simulink model "mars_rover_test_harness_chassis"  (R2025a)
settings: Solver=ode23t  StartTime=0.0  StopTime=30  FixedStep=1e-10  MaxStep=1e-1  RelTol=1e-3  AbsTol=1e-3  EnableMultiTasking=on
undefined symbols (not defined in the file): arm_q0, Control, L1, L2, L3, LS1, LS3, R1, R2, R3, Rover, RS1, RS3, X, Y, Z
libraries: sm_lib x119, nesl_utility x99, fl_lib x85, sdl_lib x20, ee_lib x10, mars_rover_lib x8, simulink x5, slpidlib x3, batteryecm_lib x2
(part 1 of 8)
Description:
  | Mars Rover Chassis Test Harness
  | Copyright 2022-2025 The MathWorks, Inc.
settings Model: VariantFading=off  Creator=The MathWorks, Inc.  LastModifiedBy=smiller
settings SolverCC: AutoScaleAbsTol=off  MaxConsecutiveZCs=500  AlgebraicLoopSolver=TrustRegion  MinimalZcImpactIntegration=on
settings DataIOCC: MaxDataPoints=10000  SaveFormat=Array  ReturnWorkspaceOutputs=off  SignalLoggingName=logsout_mars_rover_terrain
settings OptimizationCC: ReuseModelBlockBuffer=off  LifeSpan=inf
settings DebuggingCC: UnconnectedInputMsg=warning  UnconnectedOutputMsg=warning  UnconnectedLineMsg=warning  AllowSymbolicDim=off  SFUnexpectedBacktrackingDiag=warning  SFNoUnconditionalDefaultTransitionDiag=warning  SFExecutionAtInitializationDiag=none  ArithmeticOperatorsInVariantConditions=warning
settings ModelReferenceCC: EnableRefExpFcnMdlSchedulingChecks=on
settings SFSimCC: SimUseLocalCustomCode=off  CustomCodeUndefinedFunction=UseInterfaceOnly
settings RTWCC: RTWUseLocalCustomCode=off  GPUComputeCapability=3.5  DLArmComputeVersion=19.05
settings CodeAppCC: StateflowObjectComments=on
settings GRTTargetCC: TargetLangStandard=C89/C90 (ANSI)
settings ConfigComp: CovMetricSettings=dw  CovSaveCumulativeToWorkspaceVar=on  CovSaveSingleToWorkspaceVar=on  CovExternalEMLEnable=off  CovSFcnEnable=off
settings SimscapeCC: SimscapeLogType=all  SimscapeLogSimulationStatistics=on  SimscapeLogName=simlog_mars_rover_terrain  SimscapeLogLimitData=off  SimscapeLogDataHistory=10000.0  SimscapeOperatingPoint=sm_mars_rover_op
settings DiagnosticsConfigSet: SimMechanicsUnconnectedFramePorts=none  SimMechanicsConflictingReferenceFrames=none
settings ExplorerConfigSet: InternalSimMechanicsExplorerSettings="<ExplorerConfiguration><canonicalview>default</canonicalview><AnimationSetting><BasePlaybackSpeed>1.0</BasePlaybackSpeed><PlaybackSpeedFactor>2.0</PlaybackSpeedFactor></AnimationSetting><TilePanel><TileInfo><Tiles Columns=\"2\" Count=\"2\" Rows=\"1\"><Column Weight=\"0.5621\"/><Column Weight=\"0.4379\"/><Row Weight=\"1\"/><Tile Height=\"1\" Width=\"1\" X=\"0\" Y=\"0\"/><Tile Height=\"1\" Width=\"1\" X=\"1\" Y=\"0\"/></Tiles></TileInfo><SceneInfo><SceneViewer><BGColor><R>1</R><G>1</G><B>1</B></BGColor><Camera><DoPerspective>off</DoPerspective><Position><X>0.0384762068557005787</X><Y>-1.89513590882941751</Y><Z>0.280552334311850116</Z></Position><Center><X>0.0384762068557005787</X><Y>3.68387699789529677e-08</Y><Z>0.280552334311850116</Z></Center><Up><X>0</X><Y>-0</Y><Z>1</Z></Up><ViewLimDist>1</ViewLimDist><YLim>1.19054091853124122</YLim><XLim>1.46367727637290956</XLim></Camera></SceneViewer><SceneViewer><BGColor><R>1</R><G>1</G><B>1</B></BGColor><Camera><DoPerspective>off</DoPerspective><Position><X>0.0374473281726132104</X><Y>-0.000143741231528847491</Y><Z>2.19998367982950649</Z></Position><Center><X>0.0374473281726132104</X><Y>-0.000143741231528847491</Y><Z>0.280552368074773462</Z></Center><Up><X>0.999998749919673302</X><Y>0.00158118913824325125</Y><Z>0</Z></Up><ViewLimDist>1</ViewLimDist><YLim>1.46318539738655096</YLim><XLim>1.39912298944493307</XLim></Camera></SceneViewer></SceneInfo></TilePanel><MechEditorPanel><Cameras><Camera><Id>Camera7</Id><Value><Name>Chassis_Rear</Name><NativeCamera><PositionTrackingFeature>Rover.Chassis.Chassis.Camera_Frames.Reference_Chassis_Camera_Rear.R</PositionTrackingFeature><CenterTrackingFeature>Rover.Chassis.Chassis.Camera_Frames.Reference_Chassis_Camera_Rear.R</CenterTrackingFeature><UpVectorTrackingFeature>Rover.World_Frame.W</UpVectorTrackingFeature><CenterTrackingOrigin>off</CenterTrackingOrigin><CenterTrackingDirection>-Y</CenterTrackingDirection><UpVectorTrackingDirection>+Z</UpVectorTrackingDirection></NativeCamera></Value></Camera><Camera><Id>Camera8</Id><Value><Name>Chassis_Right</Name><NativeCamera><PositionTrackingFeature>Rover.Chassis.Chassis.Camera_Frames.Reference_Chassis_Camera_Right.R</PositionTrackingFeature><CenterTrackingFeature>Rover.Chassis.Chassis.Camera_Frames.Reference_Chassis_Camera_Right.R</CenterTrackingFeature><UpVectorTrackingFeature>Rover.World_Frame.W</UpVectorTrackingFeature><CenterTrackingOrigin>off</CenterTrackingOrigin><CenterTrackingDirection>+X</CenterTrackingDirection><UpVectorTrackingDirection>+Z</UpVectorTrackingDirection></NativeCamera></Value></Camera><Camera><Id>Camera9</Id><Value><Name>Chassis_Top</Name><NativeCamera><PositionTrackingFeature>Rover.Chassis.Chassis.Camera_Frames.Reference_Chassis_Camera_Top.R</PositionTrackingFeature><CenterTrackingFeature>Rover.Chassis.Chassis.Camera_Frames.Reference_Chassis_Camera_Top.R</CenterTrackingFeature><UpVectorTrackingFeature>Rover.World_Frame.W</UpVectorTrackingFeature><CenterTrackingOrigin>off</CenterTrackingOrigin><CenterTrackingDirection>-Z</CenterTrackingDirection><UpVectorTrackingDirection>+Y</UpVectorTrackingDirection></NativeCamera></Value></Camera><Camera><Id>Camera10</Id><Value><Name>Whl_L1</Name><NativeCamera><PositionTrackingFeature>Rover.Chassis.Roll_and_Steer.Drive.Camera_Frame_L1.Reference_Cam_Whl.R</PositionTrackingFeature><CenterTrackingFeature>Rover.Chassis.Roll_and_Steer.Drive.Camera_Frame_L1.Reference_Cam_Whl.R</CenterTrackingFeature><UpVectorTrackingFeature>Rover.Chassis.Roll_and_Steer.Drive.Camera_Frame_L1.Reference_Cam_Whl.R</UpVectorTrackingFeature><CenterTrackingOrigin>off</CenterTrackingOrigin><CenterTrackingDirection>-Z</CenterTrackingDirection><UpVectorTrackingDirection>+X</UpVectorTrackingDirection></NativeCamera></Value></Camera><Camera><Id>Camera11</Id><Value><Name>Whl_R1</Name><NativeCamera><PositionTrackingFeature>Rover.Chassis.Roll_and_Steer.Drive.Camera_Frame_R1.Reference_Cam_Whl.R</PositionTrackingFeature><CenterTrackingFeature>Rover.Chassis.Roll_and_Steer.Drive.Camera_Frame_R1.Reference_Cam_Whl.R</CenterTrackingFeature><UpVectorTrackingFeature>Rover.Chassis.Roll_and_Steer.Drive.Camera_Frame_R1.Reference_Cam_Whl.R</UpVectorTrackingFeature><CenterTrackingOrigin>off</CenterTrackingOrigin><CenterTrackingDirection>+Z</CenterTrackingDirection><UpVectorTrackingDirection>-X</UpVectorTrackingDirection></NativeCamera></Value></Camera><Camera><Id>Camera12</Id><Value><Name>Whl_L2</Name><NativeCamera><PositionTrackingFeature>Rover.Chassis.Roll_and_Steer.Drive.Camera_Frame_L2.Reference_Cam_Whl.R</PositionTrackingFeature><CenterTrackingFeature>Rover.Chassis.Roll_and_Steer.Drive.Camera_Frame_L2.Reference_Cam_Whl.R</CenterTrackingFeature><UpVectorTrackingFeature>Rover.Chassis.Roll_and_Steer.Drive.Camera_Frame_L2.Reference_Cam_Whl.R</UpVectorTrackingFeature><CenterTrackingOrigin>off</CenterTrackingOrigin><CenterTrackingDirection>-Z</CenterTrackingDirection><UpVectorTrackingDirection>-Y</UpVectorTrackingDirection></NativeCamera></Value></Camera><Camera><Id>Camera13</Id><Value><Name>Whl_R2</Name><NativeCamera><PositionTrackingFeature>Rover.Chassis.Roll_and_Steer.Drive.Camera_Frame_R2.Reference_Cam_Whl.R</PositionTrackingFeature><CenterTrackingFeature>Rover.Chassis.Roll_and_Steer.Drive.Camera_Frame_R2.Reference_Cam_Whl.R</CenterTrackingFeature><UpVectorTrackingFeature>Rover.Chassis.Roll_and_Steer.Drive.Camera_Frame_R2.Reference_Cam_Whl.R</UpVectorTrackingFeature><CenterTrackingOrigin>off</CenterTrackingOrigin><CenterTrackingDirection>+Z</CenterTrackingDirection><UpVectorTrackingDirection>+Y</UpVectorTrackingDirection></NativeCamera></Value></Camera><Camera><Id>Camera14</Id><Value><Name>Whl_L3</Name><NativeCamera><PositionTrackingFeature>Rover.Chassis.Roll_and_Steer.Drive.Camera_Frame_L3.Reference_Cam_Whl.R</PositionTrackingFeature><CenterTrackingFeature>Rover.Chassis.Roll_and_Steer.Drive.Camera_Frame_L3.Reference_Cam_Whl.R</CenterTrackingFeature><UpVectorTrackingFeature>Rover.Chassis.Roll_and_Steer.Drive.Camera_Frame_L3.Reference_Cam_Whl.R</UpVectorTrackingFeature><CenterTrackingOrigin>off</CenterTrackingOrigin><CenterTrackingDirection>-Z</CenterTrackingDirection><UpVectorTrackingDirection>+X</UpVectorTrackingDirection></NativeCamera></Value></Camera><Camera><Id>Camera15</Id><Value><Name>Whl_R3</Name><NativeCamera><PositionTrackingFeature>Rover.Chassis.Roll_and_Steer.Drive.Camera_Frame_R3.Reference_Cam_Whl.R</PositionTrackingFeature><CenterTrackingFeature>Rover.Chassis.Roll_and_Steer.Drive.Camera_Frame_R3.Reference_Cam_Whl.R</CenterTrackingFeature><UpVectorTrackingFeature>Rover.Chassis.Roll_and_Steer.Drive.Camera_Frame_R3.Reference_Cam_Whl.R</UpVectorTrackingFeature><CenterTrackingOrigin>off</CenterTrackingOrigin><CenterTrackingDirection>+Z</CenterTrackingDirection><UpVectorTrackingDirection>-X</UpVectorTrackingDirection></NativeCamera></Value></Camera><Camera><Id>Camera16</Id><Value><Name>Chassis_FR</Name><NativeCamera><PositionTrackingFeature>Rover.Chassis.Chassis.Camera_Frames.Reference_Chassis_Camera_FR.R</PositionTrackingFeature><CenterTrackingFeature>Rover.Chassis.Chassis.Camera_Frames.Reference_Chassis_Camera_FR.R</CenterTrackingFeature><UpVectorTrackingFeature>Rover.World_Frame.W</UpVectorTrackingFeature><CenterTrackingOrigin>off</CenterTrackingOrigin><CenterTrackingDirection>+X</CenterTrackingDirection><UpVectorTrackingDirection>+Z</UpVectorTrackingDirection></NativeCamera></Value></Camera><Camera><Id>Camera17</Id><Value><Name>Chassis_Front</Name><NativeCamera><PositionTrackingFeature>Rover.Chassis.Chassis.Camera_Frames.Reference_Chassis_Camera_Front.R</PositionTrackingFeature><CenterTrackingFeature>Rover.Chassis.Chassis.Camera_Frames.Reference_Chassis_Camera_Front.R</CenterTrackingFeature><UpVectorTrackingFeature>Rover.World_Frame.W</UpVectorTrackingFeature><CenterTrackingOrigin>off</CenterTrackingOrigin><CenterTrackingDirection>+X</CenterTrackingDirection><UpVectorTrackingDirection>+Z</UpVectorTrackingDirection></NativeCamera></Value></Camera><Camera><Id>Camera18</Id><Value><Name>Chassis_WhlFR</Name><NativeCamera><PositionTrackingFeature>Rover.Chassis.Chassis.Camera_Frames.Reference_Chassis_Camera_WhlFR.R</PositionTrackingFeature><CenterTrackingFeature>Rover.Chassis.Chassis.Camera_Frames.Reference_Chassis_Camera_WhlFR.R</CenterTrackingFeature><UpVectorTrackingFeature>Rover.World_Frame.W</UpVectorTrackingFeature><CenterTrackingOrigin>off</CenterTrackingOrigin><CenterTrackingDirection>+X</CenterTrackingDirection><UpVectorTrackingDirection>+Z</UpVectorTrackingDirection></NativeCamera></Value></Camera><Camera><Id>Camera19</Id><Value><Name>Chassis_WhlRR</Name><NativeCamera><PositionTrackingFeature>Rover.Chassis.Chassis.Camera_Frames.Reference_Chassis_Camera_WhlRR.R</PositionTrackingFeature><CenterTrackingFeature>Rover.Chassis.Chassis.Camera_Frames.Reference_Chassis_Camera_WhlRR.R</CenterTrackingFeature><UpVectorTrackingFeature>Rover.World_Frame.W</UpVectorTrackingFeature><CenterTrackingOrigin>off</CenterTrackingOrigin><CenterTrackingDirection>+X</CenterTrackingDirection><UpVectorTrackingDirection>+Z</UpVectorTrackingDirection></NativeCamera></Value></Camera><Camera><Id>Camera20</Id><Value><Name>Chassis_Camera_Lens</Name><NativeCamera><PositionTrackingFeature>Rover.Chassis.Camera.rsm_head_1_RIGID.Reference_Camera.R</PositionTrackingFeature><CenterTrackingFeature>Rover.Chassis.Camera.rsm_head_1_RIGID.Reference_Camera.R</CenterTrackingFeature><UpVectorTrackingFeature>Rover.Chassis.Camera.rsm_head_1_RIGID.Reference_Camera.R</UpVectorTrackingFeature><CenterTrackingOrigin>off</CenterTrackingOrigin><CenterTrackingDirection>+Z</CenterTrackingDirection><UpVectorTrackingDirection>+X</UpVectorTrackingDirection></NativeCamera></Value></Camera></Cameras><GfxPanelCameraMap/><VideoCreator><PlaybackSpeedRatio>1.0</PlaybackSpeedRatio><FrameRate>30</FrameRate><VideoFormat>MPEG-4</VideoFormat><FrameSize>auto</FrameSize></VideoCreator></MechEditorPanel></ExplorerConfiguration>"

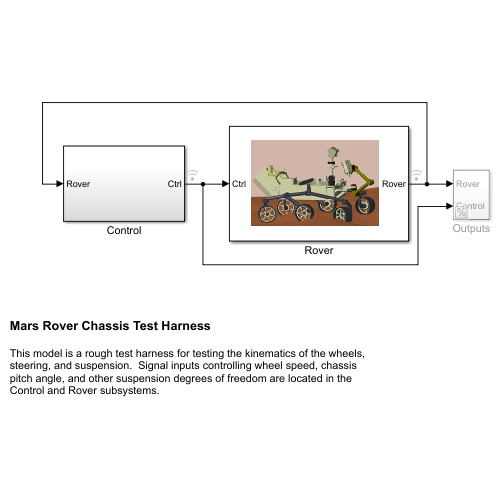
[thumbnail: Simulink's stored preview of the top-level diagram]
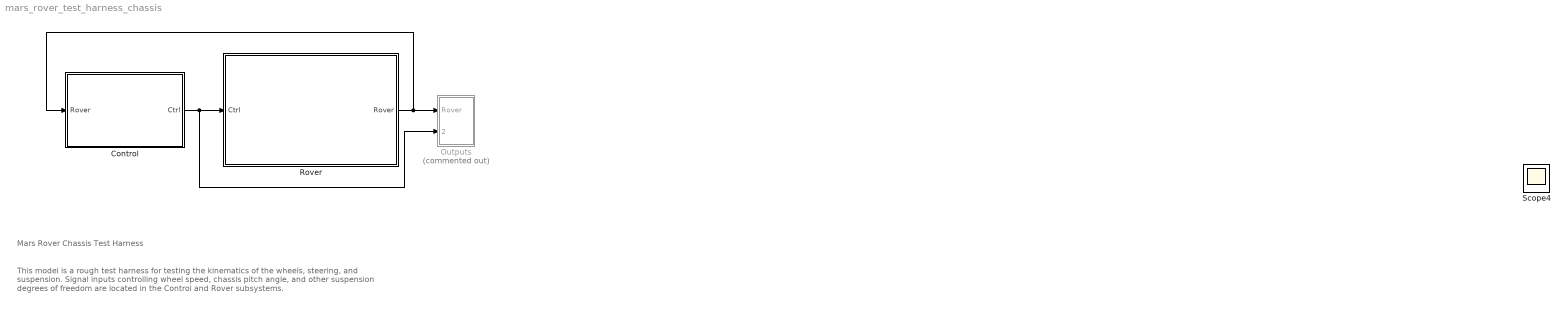
== system mars_rover_test_harness_chassis ==
  note: This model is a rough test harness for testing the kinematics of the wheels, steering, and suspension. Signal inputs controlling wheel speed, chassis pitch angle, and other suspension degrees of freedom are located in the Control and Rover subsystems.
  note: Mars Rover Chassis Test Harness
  Control : Subsystem
  Outputs : Subsystem  Commented=on
  Rover : Subsystem
      mask Display: image('mars_rover_terrain_rover.png')
  Scope4 : Scope
      settings: ActiveDisplayYMinimum=-0.1776  ActiveDisplayYMaximum=0.10656  DataLoggingVariableName=ScopeData5
  wires:
  Control/1(Ctrl) -> Outputs/2(Control), Rover/1(Ctrl)
  Rover/1(Rover) -> Control/1(Rover), Outputs/1(Rover)

== system mars_rover_test_harness_chassis/Control ==
  In Bus Element : Inport  PortName=Rover  Element=Arm
  In Bus Element1 : Inport  PortName=Rover  Element=Chassis
  Arm Control : Subsystem
  Chassis Control : Subsystem
  Out Bus Element : Outport  PortName=Ctrl  Element=Arm
  Out Bus Element1 : Outport  PortName=Ctrl  Element=Chassis
  wires:
  Arm Control/1(Ctrl) -> Out Bus Element/1
  Chassis Control/1(Ctrl) -> Out Bus Element1/1
  In Bus Element/1 -> Arm Control/1(Arm)
  In Bus Element1/1 -> Chassis Control/1(Chassis)

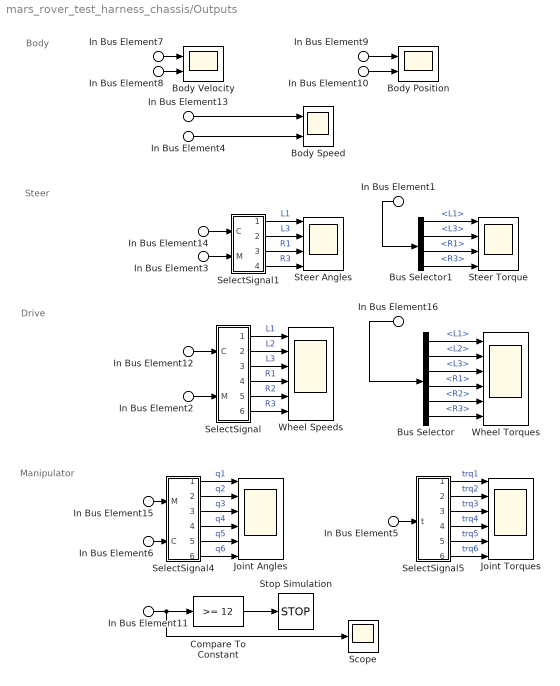
== system mars_rover_test_harness_chassis/Outputs ==
  note: Body
  note: Steer
  note: Drive
  note: Manipulator
  In Bus Element2 : Inport  PortName=Rover  Element=Chassis.Wheels.Drive
  In Bus Element16 : Inport  PortName=Rover  Element=Chassis.Wheels.Drive.trq
  In Bus Element3 : Inport  PortName=Rover  Element=Chassis.Wheels.Steer
  In Bus Element15 : Inport  PortName=Rover  Element=Arm.q
  In Bus Element7 : Inport  PortName=Rover  Element=Body.vxy
  In Bus Element8 : Inport  PortName=Rover  Element=Body.wz
  In Bus Element9 : Inport  PortName=Rover  Element=Body.xyz
  In Bus Element10 : Inport  PortName=Rover  Element=Body.rpy
  In Bus Element4 : Inport  PortName=Rover  Element=Body.v
  In Bus Element1 : Inport  Port=2  PortName=Control  Element=Chassis.Steer
  In Bus Element12 : Inport  Port=2  PortName=Control  Element=Chassis.Cmd.wWhl
  In Bus Element13 : Inport  Port=2  PortName=Control  Element=Chassis.Cmd.v
  In Bus Element14 : Inport  Port=2  PortName=Control  Element=Chassis.Cmd.qSteer
  In Bus Element5 : Inport  Port=2  PortName=Control  Element=Arm.trq
  In Bus Element6 : Inport  Port=2  PortName=Control  Element=Arm.qCmd
  In Bus Element11 : Inport  Port=2  PortName=Control  Element=Arm.Mode
  Body Position : Scope  NumInputPorts=2
      settings: Title=Rover Position and Orientation  ActiveDisplayYMinimum=-4.54452  ActiveDisplayYMaximum=67.13718  YLabel=Rover XYZ Position (m)  DataLoggingVariableName=ScopeData2
  Body Speed : Scope  NumInputPorts=2
      settings: ActiveDisplayYMinimum=-0.02002  ActiveDisplayYMaximum=0.33686  DataLoggingVariableName=ScopeData7
  Body Velocity : Scope  NumInputPorts=2
      settings: Title=Rover Linear and Ang Velocities  ActiveDisplayYMinimum=-0.35082  ActiveDisplayYMaximum=0.38387  YLabel=Rover Linear Vel (m/s)
  Bus Selector : BusSelector  OutputSignals=L1,L2,L3,R1,R2,R3
  Bus Selector1 : BusSelector  OutputSignals=trq.L1,trq.L3,trq.R1,trq.R3
  Compare To Constant : simulink/Logic and Bit Operations/Compare To Constant  relop=>=  const=12  OutDataTypeStr=boolean
  Joint Angles : Scope  NumInputPorts=6
      settings: Title=Joint 1  ActiveDisplayYMinimum=-13.90292  ActiveDisplayYMaximum=99.39774  YLabel=Joint Angle (deg)  DataLoggingVariableName=ScopeData2
  Joint Torques : Scope  NumInputPorts=6
      settings: Title=Joint 1  ActiveDisplayYMinimum=-1231.55572  ActiveDisplayYMaximum=1377.74123  YLabel=Torque (N*m)
  Scope : Scope
      settings: ActiveDisplayYMinimum=-1.5  ActiveDisplayYMaximum=13.5
  SelectSignal : Subsystem
  SelectSignal1 : Subsystem
  SelectSignal4 : Subsystem
  SelectSignal5 : Subsystem
  Steer Angles : Scope  NumInputPorts=4
      settings: ActiveDisplayYMinimum=-23.51402  ActiveDisplayYMaximum=36.5986  YLabel=Steer Angle (Deg)  DataLoggingVariableName=ScopeData3
  Steer Torque : Scope  NumInputPorts=4
      settings: ActiveDisplayYMinimum=-139.38584  ActiveDisplayYMaximum=135.19843  YLabel=Torque (N*m)  DataLoggingVariableName=ScopeData4
  Stop Simulation : Stop
  Wheel Speeds : Scope  NumInputPorts=6
      settings: ActiveDisplayYMinimum=-0.5  ActiveDisplayYMaximum=4  YLabel=Wheel Speed (rad/s)  DataLoggingVariableName=ScopeData5
  Wheel Torques : Scope  NumInputPorts=6
      settings: ActiveDisplayYMinimum=17.86848  ActiveDisplayYMaximum=20.11099  YLabel=Torque (N*m)  DataLoggingVariableName=ScopeData6
  wires:
  In Bus Element4/1 -> Body Speed/2
  In Bus Element8/1 -> Body Velocity/2
  In Bus Element7/1 -> Body Velocity/1
  In Bus Element16/1 -> Bus Selector/1
  SelectSignal1/2(L3) -> Steer Angles/2  "L3"
  In Bus Element9/1 -> Body Position/1
  Bus Selector/3 -> Wheel Torques/3  "<L3>"
  In Bus Element10/1 -> Body Position/2
  Bus Selector/6 -> Wheel Torques/6  "<R3>"
  SelectSignal/3(L3) -> Wheel Speeds/3  "L3"
  SelectSignal/1(L1) -> Wheel Speeds/1  "L1"
  SelectSignal/6(R3) -> Wheel Speeds/6  "R3"
  Bus Selector/1 -> Wheel Torques/1  "<L1>"
  SelectSignal1/4(R3) -> Steer Angles/4  "R3"
  SelectSignal/2(L2) -> Wheel Speeds/2  "L2"
  SelectSignal/5(R2) -> Wheel Speeds/5  "R2"
  Bus Selector/2 -> Wheel Torques/2  "<L2>"
  SelectSignal/4(R1) -> Wheel Speeds/4  "R1"
  SelectSignal1/1(L1) -> Steer Angles/1  "L1"
  SelectSignal1/3(R1) -> Steer Angles/3  "R1"
  In Bus Element13/1 -> Body Speed/1
  Bus Selector/4 -> Wheel Torques/4  "<R1>"
  Bus Selector/5 -> Wheel Torques/5  "<R2>"
  In Bus Element1/1 -> Bus Selector1/1
  Bus Selector1/1 -> Steer Torque/1  "<L1>"
  Bus Selector1/2 -> Steer Torque/2  "<L3>"
  Bus Selector1/3 -> Steer Torque/3  "<R1>"
  Bus Selector1/4 -> Steer Torque/4  "<R3>"
  In Bus Element2/1 -> SelectSignal/2(M)
  In Bus Element3/1 -> SelectSignal1/2(M)
  In Bus Element5/1 -> SelectSignal5/1(t)
  SelectSignal4/1(q1) -> Joint Angles/1  "q1"
  In Bus Element15/1 -> SelectSignal4/1(M)
  SelectSignal5/1(t1) -> Joint Torques/1  "trq1"
  SelectSignal5/4(t4) -> Joint Torques/4  "trq4"
  SelectSignal4/4(q4) -> Joint Angles/4  "q4"
  SelectSignal4/2(q2) -> Joint Angles/2  "q2"
  SelectSignal5/5(t5) -> Joint Torques/5  "trq5"
  SelectSignal5/3(t3) -> Joint Torques/3  "trq3"
  SelectSignal5/2(t2) -> Joint Torques/2  "trq2"
  SelectSignal5/6(t6) -> Joint Torques/6  "trq6"
  SelectSignal4/3(q3) -> Joint Angles/3  "q3"
  SelectSignal4/6(q6) -> Joint Angles/6  "q6"
  SelectSignal4/5(q5) -> Joint Angles/5  "q5"
  In Bus Element6/1 -> SelectSignal4/2(C)
  In Bus Element12/1 -> SelectSignal/1(C)
  In Bus Element14/1 -> SelectSignal1/1(C)
  In Bus Element11/1 -> Scope/1, Compare To Constant/1
  Compare To Constant/1 -> Stop Simulation/1

== system mars_rover_test_harness_chassis/Rover ==
  In Bus Element : Inport  PortName=Ctrl  Element=Arm.trq
  In Bus Element3 : Inport  PortName=Ctrl  Element=Chassis
  Arm : mars_rover_lib/Arm  arm_q0_deg=arm_q0
  Chassis : Subsystem
      settings: PortSchema="{\"entries\":[{\"content\":{\"sides\":[{\"content\":{\"connectorIds\":[\"LConn1\",\"LConn2\",\"In1\",\"LConn3\",\"LConn4\"]},\"type\":\"ConnectorPlacement.EquallySpacedRectSide\",\"uuid\":\"1e8a3e2b-b3ca-4467-863a-9c237d71771f\"},{\"content\":{\"connectorIds\":[\"Out1\"],\"side\":\"RIGHT\"},\"type\":\"ConnectorPlacement.EquallySpacedRectSide\",\"uuid\":\"1c304fdb-ff64-4dc8-bd28-208b239a200a\"},{\"content\":{\"connectorIds\":[],\"side\":\"TOP\"},\"type\":\"ConnectorPlacement.EquallySpacedRectSide\",\"uuid\":\"6fd19973-5814-4525-bce6-20dd9c942e44\"}]},\"type\":\"ConnectorPlacement.EquallySpacedConnector\",\"uuid\":\"720db96a-3f3b-4ddd-a986-ea75ab459e47\"}],\"packageUris\":[\"http://schema.mathworks.com/mf0/Connector/R2020b\"],\"version\":\"1.0\"}"
      mask Display: image('mars_rover_terrain_chassis.png');
  Mechanism Configuration : sm_lib/Utilities/Mechanism Configuration  UniformGravity=Constant  GravityVector=[0 0 -3.72076]  GravityVectorUnits=m/s^2  LinearizationDelta=0.001  JointModeTransitionNonlinearIterations=2
  Set Body Pitch : Subsystem
  Solver Configuration : nesl_utility/Solver Configuration  PhysicalDomain=network_engine_domain  SubClassName=solver  LeftPortType=input  RightPortType=generic  Tones=[]  Harmonics=[]  SimulateNoise=off  Profile=off  UseLocalSampling=off  EnableSwitchedLinearOptims=on  FrequencyDomain=off  UseCCode=off  RelTol=0.001  AbsTol=1e-06  MinStep=1e-09  ToWorkspace=off  RevertToSquareIcSolve=off  NumHomotopyIterations=100  PhasorMode=off  PhasorModeNumHarmonics=1  ConsistencySolver=NEWTON_FTOL  IndexReductionMethod=DerivativeReplacement  DoDC=off  ResidualTolerance=1e-09  ConsistencyTolSource=GLOBAL  ConsistencyAbsTol=0.001  ConsistencyRelTol=0.001  ConsistencyTolFactor=0.001  UseLocalSolver=off  LocalSolverChoice=NE_BACKWARD_EULER_ADVANCER  ResolveIndetEquations=on  FunctionEvalNumThread=1  LocalSolverSampleTime=0.001  DoFixedCost=off  MaxNonlinIter=3  MaxModeIter=2  ComputeImpulses=off  ImpulseIterations=2  LinearAlgebra=auto  LinearAlgebraNumThread=0  EquationFormulation=NE_TIME_EF  DelaysMemoryBudget=1024  AutomaticFiltering=on  FilteringTimeConstant=0.001  PartitionStorageMethod=AS_NEEDED  PartitionMemoryBudget=1024  PartitionMethod=FAST  MultibodyUseLocalSolver=off  MultibodyLocalSolverChoice=ODE1  MultibodyLocalSolverSampleTime=0.001
  World Frame : sm_lib/Frames and Transforms/World Frame
  Out Bus Element : Outport  PortName=Rover  Element=Arm
  Out Bus Element1 : Outport  PortName=Rover  Element=Chassis
  wires:
  In Bus Element/1 -> Arm/1
  In Bus Element3/1 -> Chassis/1(Ctrl)
  Arm/1 -> Out Bus Element/1
  Chassis/1(m) -> Out Bus Element1/1
  connections:
  Arm/LConn2 -- Chassis/LConn1
  Set Body Pitch/LConn1 -- World Frame/RConn1 -- Mechanism Configuration/RConn1 -- Solver Configuration/RConn1
  Set Body Pitch/RConn1 -- Chassis/LConn3

== system mars_rover_test_harness_chassis/Control/Arm Control ==
  note: Locks arm in docked position.
  In Bus Element1 : Inport  PortName=Arm
  Add : Sum  Inputs=+-
  Bus Creator : BusCreator  Inputs=3
  Bus to Vec q : Subsystem
  Constant{,1..3} (4 alike) : Constant  Value=0
  PID Control : slpidlib/PID Controller  Controller=PID  Form=Parallel  TimeDomain=Continuous-time  UseExternalTs=off  SampleTime=-1  IntegratorMethod=Forward Euler  FilterMethod=Forward Euler  ControllerParametersSource=internal  P=Control.Arm.Kp  I=Control.Arm.Ki  UseKiTs=off  D=Control.Arm.Kd  UseExternalDerivativeSource=off  N=Control.Arm.N  UseFilter=on  TunerSelectOption=Transfer Function Based (PID Tuner App)  InitialConditionSource=internal  InitialConditionForIntegrator=0  InitialConditionForFilter=0  DifferentiatorICPrevScaledInput=0  ExternalReset=none  TrackingMode=off  Kt=1  LimitOutput=off  SatLimitsSource=internal  UpperSaturationLimit=inf  LowerSaturationLimit=-inf  LinearizeAsGain=on  AntiWindupMode=none  Kb=1  LimitIntegrator=off  UpperIntegratorSaturationLimit=inf  LowerIntegratorSaturationLimit=-inf  POutMin=[]  POutMax=[]  IOutMin=[]  IOutMax=[]  DOutMin=[]  DOutMax=[]  NOutMin=[]  NOutMax=[]  SumOutMin=[]  SumOutMax=[]  SaturationOutMin=[]  SaturationOutMax=[]  PParamMin=[]  PParamMax=[]  IParamMin=[]  IParamMax=[]  DParamMin=[]  DParamMax=[]  NParamMin=[]  NParamMax=[]  KbParamMin=[]  KbParamMax=[]  KtParamMin=[]  KtParamMax=[]  KbOutMin=[]  KbOutMax=[]  KtOutMin=[]  KtOutMax=[]  IntegratorOutMin=[]  IntegratorOutMax=[]  FilterOutMin=[]  FilterOutMax=[]  SumI1OutMin=[]  SumI1OutMax=[]  SumI2OutMin=[]  SumI2OutMax=[]  SumI3OutMin=[]  SumI3OutMax=[]  SumI4OutMin=[]  SumI4OutMax=[]  SumDOutMin=[]  SumDOutMax=[]  DifferentiatorOutMin=[]  DifferentiatorOutMax=[]  FilterDiffOutCoefMin=[]  FilterDiffOutCoefMax=[]  ReciprocalOutMin=[]  ReciprocalOutMax=[]  SumDenOutMin=[]  SumDenOutMax=[]  SumNumOutMin=[]  SumNumOutMax=[]  DivideOutMin=[]  DivideOutMax=[]  UdiffTsProdOutMin=[]  UdiffTsProdOutMax=[]  NTsProdOutMin=[]  NTsProdOutMax=[]  UintegralTsProdOutMin=[]  UintegralTsProdOutMax=[]  UngainTsProdOutMin=[]  UngainTsProdOutMax=[]  ClampingZeroOutDataTypeStr=Inherit: Inherit via back propagation  ClampingZeroOutMin=[]  ClampingZeroOutMax=[]  FilterDenConstantOutDataTypeStr=Inherit: Inherit via back propagation  FilterDenConstantOutMin=[]  FilterDenConstantOutMax=[]  PCopyOutDataTypeStr=Inherit: Inherit via back propagation  PCopyOutMin=[]  PCopyOutMax=[]  NCopyOutDataTypeStr=Inherit: Inherit via back propagation  NCopyOutMin=[]  NCopyOutMax=[]  IntegratorContinuousStateAttributes=''  IntegratorStateMustResolveToSignalObject=off  IntegratorRTWStateStorageClass=Auto  FilterContinuousStateAttributes=''  FilterStateMustResolveToSignalObject=off  FilterRTWStateStorageClass=Auto  ParallelPVariant=InternalParameters  IdealPVariant=Disabled  IVariant=InternalParameters  DVariant=InternalParameters  IntegratorVariant=Continuous  SatVariant=Disabled  AWVariant=Passthrough  PCopyVariant=Disabled  TRVariant=Disabled  FdbkBlocksVariant=Forward  IdealPFdbkVariant=Disabled  SatFdbkVariant=Disabled  DerivativeFilterVariant=ContFilter  NVariant=InternalParameters  NCopyVariant=Disabled  FilterICVariant=InternalICsFilter  IntegratorICVariant=InternalICs  ExternalResetVariant=Disabled  TRSumVariant=Passthrough  SumFdbkVariant=Disabled  SumVariant=Sum_PID  TsampFilterVariant=InternalTs  TsampNgainVariant=Passthrough  TsampIntegralVariant=Disabled_SignalSpec  ExternalSaturationOutDataTypeStr=Inherit: Same as second input  DerivativeSourceVariant=ErrorSignal  PreIntVariant=InternalPreInt
  Terminator : Terminator
  Vec to Bus q : Subsystem
  Vec to Bus trq : Subsystem
  q0 Arm : Constant  Value=arm_q0
  Bus Element Out : Outport  PortName=Ctrl  Element=trq
  Out Bus Element : Outport  PortName=Ctrl  Element=Sample
  Out Bus Element1 : Outport  PortName=Ctrl  Element=qCmd
  Bus Element Out1 : Outport  PortName=Ctrl  Element=Mode
  wires:
  q0 Arm/1 -> Vec to Bus q/1(V), Add/1
  PID Control/1 -> Vec to Bus trq/1(V)
  Bus to Vec q/1(V) -> Terminator/1, Add/2
  Add/1 -> PID Control/1
  Constant/1 -> Bus Creator/1  "Hold"
  Constant1/1 -> Bus Creator/2  "Stored"
  Vec to Bus trq/1(B) -> Bus Element Out/1
  Bus Creator/1 -> Out Bus Element/1
  Vec to Bus q/1(B) -> Out Bus Element1/1
  In Bus Element1/1 -> Bus to Vec q/1(B)
  Constant3/1 -> Bus Element Out1/1
  Constant2/1 -> Bus Creator/3  "Location"

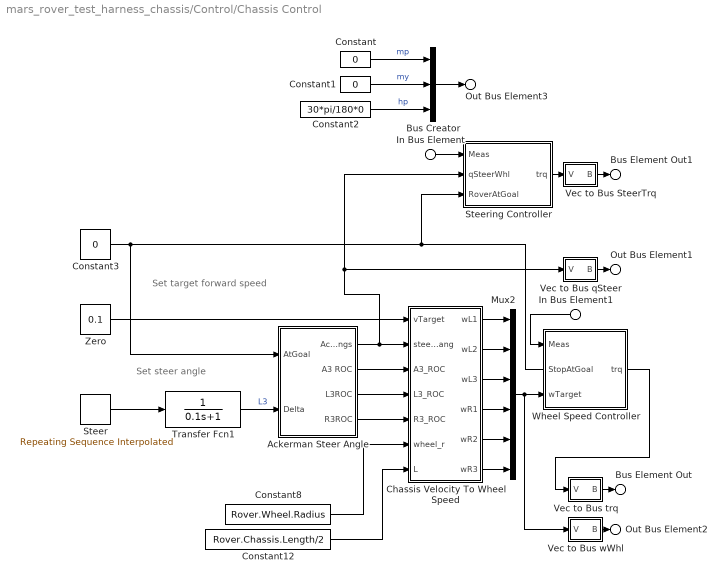
== system mars_rover_test_harness_chassis/Control/Chassis Control ==
  note: Set target forward speed
  note: Set steer angle
  In Bus Element1 : Inport  PortName=Chassis  Element=Wheels.Drive
  In Bus Element : Inport  PortName=Chassis  Element=Wheels.Steer
  Ackerman Steer Angle : Subsystem
  Bus Creator : BusCreator  Inputs=3
  Chassis Velocity To Wheel Speed : MATLAB Function  TreatAsAtomicUnit=on
  Constant : Constant  Value=0
  Constant1 : Constant  Value=0
  Constant12 : Constant  Value=Rover.Chassis.Length/2
  Constant2 : Constant  Value=30*pi/180*0
  Constant3 : Constant  Value=0
  Constant8 : Constant  Value=Rover.Wheel.Radius
  Mux2 : Mux  Inputs=6
  Steer : simulink/Sources/Repeating Sequence Interpolated  OutValues=[0 0 1 1 0 0 -1 -1 0 0]*30.'  TimeValues=[0 2 4 7+5 9+5 11+5 13+5 16+10 18+10 20+10].'  LookUpMeth=Interpolation-Use End Values  tsamp=0.01  OutMin=[]  OutMax=[]  OutDataTypeStr=double  OutputDataTypeScalingMode=double  OutDataType=fixdt(0,8)  OutScaling=2^-10
  Steering Controller : Subsystem  mask{Kp=Control.Steer.Kp, Ki=Control.Steer.Ki, Kd=Control.Steer.Kd, N=Control.Steer.N, Ts_Targetq=Control.Steer.FiltTargetq, Ts_Measq=Control.Steer.FiltSensorq, trq_max_pos=Control.Steer.TrqCmdLimitPos, trq_max_neg=Control.Steer.TrqCmdLimitNeg}
      mask prompts: Kp "Propotional Gain"; Ki "Integral Gain"; Kd "Derivative Gain"; N "Filter Constant (derivative)"; Ts_Targetq "Target Angle (deg)"; Ts_Measq "Sensed Angle (deg)"; trq_max_pos "Torque Command Upper Limit (N*m)"; trq_max_neg "Torque Command Lower Limit (N*m)"
      mask DialogControl cont_pid Prompt: PID Controller
      mask DialogControl cont_filt_ts Prompt: Filter Time Constants
      mask DialogControl cont_trqCmdLim Prompt: Limits at Wheel
  Transfer Fcn1 : TransferFcn  Denominator=[0.1 1]
  Vec to Bus SteerTrq : Subsystem
  Vec to Bus qSteer : Subsystem
  Vec to Bus trq : Subsystem
  Vec to Bus wWhl : Subsystem
  Wheel Speed Controller : Subsystem  mask{Kp=Control.Drive.Kp, Ki=Control.Drive.Ki, Kd=Control.Drive.Kd, N=Control.Drive.N, Ts_Targetw=Control.Drive.FiltTargetw, Ts_Measw=Control.Drive.FiltSensorw, trq_max_pos=Control.Drive.TrqCmdLimitPos, trq_max_neg=Control.Drive.TrqCmdLimitNeg}
      mask prompts: Kp "Propotional Gain"; Ki "Integral Gain"; Kd "Derivative Gain"; N "Filter Constant (derivative)"; Ts_Targetw "Target Speed (sec)"; Ts_Measw "Sensed Speed (sec)"; trq_max_pos "Torque Command Upper Limit (N*m)"; trq_max_neg "Torque Command Lower Limit (N*m)"
      mask DialogControl Container4 Prompt: PID Controller
      mask DialogControl cont_filt_ts Prompt: Filter Time Constants
      mask DialogControl cont_trqCmdLim Prompt: Limits
  Zero : Constant  Value=0.1  OutDataTypeStr=Inherit: Inherit via back propagation
  Bus Element Out1 : Outport  PortName=Ctrl  Element=Steer.trq
  Bus Element Out : Outport  PortName=Ctrl  Element=Drive.trq
  Out Bus Element1 : Outport  PortName=Ctrl  Element=Cmd.qSteer
  Out Bus Element2 : Outport  PortName=Ctrl  Element=Cmd.wWhl
  Out Bus Element3 : Outport  PortName=Ctrl  Element=Camera
  wires:
  Mux2/1 -> Wheel Speed Controller/3(wTarget), Vec to Bus wWhl/1(V)
  Wheel Speed Controller/1(trq) -> Vec to Bus trq/1(V)
  Steering Controller/1(trq) -> Vec to Bus SteerTrq/1(V)
  Vec to Bus trq/1(B) -> Bus Element Out/1
  Vec to Bus SteerTrq/1(B) -> Bus Element Out1/1
  In Bus Element1/1 -> Wheel Speed Controller/1(Meas)
  In Bus Element/1 -> Steering Controller/1(Meas)
  Vec to Bus qSteer/1(B) -> Out Bus Element1/1
  Vec to Bus wWhl/1(B) -> Out Bus Element2/1
  Constant3/1 -> Ackerman Steer Angle/1(AtGoal), Wheel Speed Controller/2(StopAtGoal), Steering Controller/3(RoverAtGoal)
  Constant/1 -> Bus Creator/1  "mp"
  Constant1/1 -> Bus Creator/2  "my"
  Constant2/1 -> Bus Creator/3  "hp"
  Bus Creator/1 -> Out Bus Element3/1
  Ackerman Steer Angle/1(AckSteerAngs) -> Steering Controller/2(qSteerWhl), Vec to Bus qSteer/1(V), Chassis Velocity To Wheel Speed/2(steer_ang)
  Steer/1 -> Transfer Fcn1/1
  Transfer Fcn1/1 -> Ackerman Steer Angle/2(Delta)  "L3"
  Ackerman Steer Angle/2(A3 ROC) -> Chassis Velocity To Wheel Speed/3(A3_ROC)
  Ackerman Steer Angle/3(L3ROC) -> Chassis Velocity To Wheel Speed/4(L3_ROC)
  Ackerman Steer Angle/4(R3ROC) -> Chassis Velocity To Wheel Speed/5(R3_ROC)
  Constant12/1 -> Chassis Velocity To Wheel Speed/7(L)
  Constant8/1 -> Chassis Velocity To Wheel Speed/6(wheel_r)
  Chassis Velocity To Wheel Speed/1(wL1) -> Mux2/1
  Chassis Velocity To Wheel Speed/2(wL2) -> Mux2/2
  Chassis Velocity To Wheel Speed/3(wL3) -> Mux2/3
  Chassis Velocity To Wheel Speed/4(wR1) -> Mux2/4
  Chassis Velocity To Wheel Speed/5(wR2) -> Mux2/5
  Chassis Velocity To Wheel Speed/6(wR3) -> Mux2/6
  Zero/1 -> Chassis Velocity To Wheel Speed/1(vTarget)

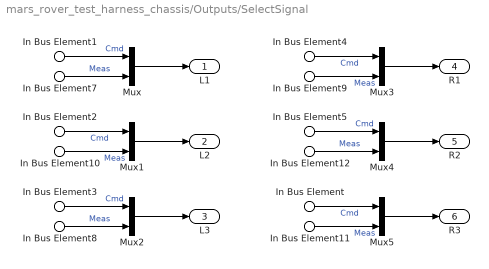
== system mars_rover_test_harness_chassis/Outputs/SelectSignal ==
  In Bus Element1 : Inport  PortName=C  Element=L1
  In Bus Element2 : Inport  PortName=C  Element=L2
  In Bus Element3 : Inport  PortName=C  Element=L3
  In Bus Element4 : Inport  PortName=C  Element=R1
  In Bus Element5 : Inport  PortName=C  Element=R2
  In Bus Element : Inport  PortName=C  Element=R3
  In Bus Element7 : Inport  Port=2  PortName=M  Element=w.L1
  In Bus Element10 : Inport  Port=2  PortName=M  Element=w.L2
  In Bus Element8 : Inport  Port=2  PortName=M  Element=w.L3
  In Bus Element11 : Inport  Port=2  PortName=M  Element=w.R3
  In Bus Element12 : Inport  Port=2  PortName=M  Element=w.R2
  In Bus Element9 : Inport  Port=2  PortName=M  Element=w.R1
  Mux{,1..5} (6 alike) : Mux  Inputs=2
  L1 : Outport
  L2 : Outport  Port=2
  L3 : Outport  Port=3
  R1 : Outport  Port=4
  R2 : Outport  Port=5
  R3 : Outport  Port=6
  wires:
  In Bus Element7/1 -> Mux/2  "Meas"
  Mux/1 -> L1/1
  In Bus Element1/1 -> Mux/1  "Cmd"
  In Bus Element2/1 -> Mux1/1  "Cmd"
  Mux1/1 -> L2/1
  In Bus Element10/1 -> Mux1/2  "Meas"
  In Bus Element8/1 -> Mux2/2  "Meas"
  Mux2/1 -> L3/1
  In Bus Element3/1 -> Mux2/1  "Cmd"
  In Bus Element4/1 -> Mux3/1  "Cmd"
  Mux3/1 -> R1/1
  In Bus Element9/1 -> Mux3/2  "Meas"
  In Bus Element12/1 -> Mux4/2  "Meas"
  Mux4/1 -> R2/1
  In Bus Element5/1 -> Mux4/1  "Cmd"
  In Bus Element/1 -> Mux5/1  "Cmd"
  Mux5/1 -> R3/1
  In Bus Element11/1 -> Mux5/2  "Meas"

== system mars_rover_test_harness_chassis/Outputs/SelectSignal1 ==
  In Bus Element1 : Inport  PortName=C  Element=L1
  In Bus Element3 : Inport  PortName=C  Element=L3
  In Bus Element4 : Inport  PortName=C  Element=R3
  In Bus Element2 : Inport  PortName=C  Element=R1
  In Bus Element5 : Inport  Port=2  PortName=M  Element=q.L1
  In Bus Element6 : Inport  Port=2  PortName=M  Element=q.L3
  In Bus Element7 : Inport  Port=2  PortName=M  Element=q.R1
  In Bus Element8 : Inport  Port=2  PortName=M  Element=q.R3
  Mux{,1..3} (4 alike) : Mux  Inputs=2
  L1 : Outport
  L3 : Outport  Port=2
  R1 : Outport  Port=3
  R3 : Outport  Port=4
  wires:
  In Bus Element8/1 -> Mux3/2  "Meas"
  Mux3/1 -> R3/1
  In Bus Element2/1 -> Mux2/1  "Cmd"
  In Bus Element4/1 -> Mux3/1  "Cmd"
  Mux2/1 -> R1/1
  In Bus Element7/1 -> Mux2/2  "Meas"
  In Bus Element6/1 -> Mux1/2  "Meas"
  Mux1/1 -> L3/1
  In Bus Element1/1 -> Mux/1  "Cmd"
  In Bus Element3/1 -> Mux1/1  "Cmd"
  Mux/1 -> L1/1
  In Bus Element5/1 -> Mux/2  "Meas"

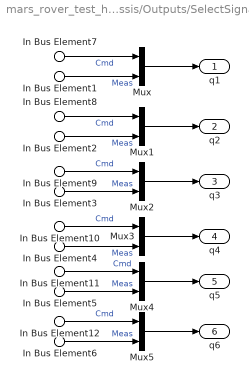
== system mars_rover_test_harness_chassis/Outputs/SelectSignal4 ==
  In Bus Element1 : Inport  PortName=M  Element=q1
  In Bus Element2 : Inport  PortName=M  Element=q2
  In Bus Element3 : Inport  PortName=M  Element=q3
  In Bus Element4 : Inport  PortName=M  Element=q4
  In Bus Element5 : Inport  PortName=M  Element=q5
  In Bus Element6 : Inport  PortName=M  Element=q6
  In Bus Element7 : Inport  Port=2  PortName=C  Element=q1
  In Bus Element8 : Inport  Port=2  PortName=C  Element=q2
  In Bus Element9 : Inport  Port=2  PortName=C  Element=q3
  In Bus Element10 : Inport  Port=2  PortName=C  Element=q4
  In Bus Element11 : Inport  Port=2  PortName=C  Element=q5
  In Bus Element12 : Inport  Port=2  PortName=C  Element=q6
  Mux{,1..5} (6 alike) : Mux  Inputs=2
  q1 : Outport
  q2 : Outport  Port=2
  q3 : Outport  Port=3
  q4 : Outport  Port=4
  q5 : Outport  Port=5
  q6 : Outport  Port=6
  wires:
  In Bus Element6/1 -> Mux5/2  "Meas"
  Mux5/1 -> q6/1
  In Bus Element12/1 -> Mux5/1  "Cmd"
  In Bus Element11/1 -> Mux4/1  "Cmd"
  Mux4/1 -> q5/1
  In Bus Element5/1 -> Mux4/2  "Meas"
  In Bus Element4/1 -> Mux3/2  "Meas"
  Mux3/1 -> q4/1
  In Bus Element10/1 -> Mux3/1  "Cmd"
  In Bus Element9/1 -> Mux2/1  "Cmd"
  Mux2/1 -> q3/1
  Mux1/1 -> q2/1
  In Bus Element8/1 -> Mux1/1  "Cmd"
  In Bus Element7/1 -> Mux/1  "Cmd"
  Mux/1 -> q1/1
  In Bus Element1/1 -> Mux/2  "Meas"
  In Bus Element2/1 -> Mux1/2  "Meas"
  In Bus Element3/1 -> Mux2/2  "Meas"

== system mars_rover_test_harness_chassis/Outputs/SelectSignal5 ==
  t : Inport
  Bus Selector : BusSelector  OutputSignals=t1,t2,t3,t4,t5,t6
  t1 : Outport
  t2 : Outport  Port=2
  t3 : Outport  Port=3
  t4 : Outport  Port=4
  t5 : Outport  Port=5
  t6 : Outport  Port=6
  wires:
  Bus Selector/1 -> t1/1  "<t1>"
  Bus Selector/2 -> t2/1  "<t2>"
  Bus Selector/3 -> t3/1  "<t3>"
  Bus Selector/4 -> t4/1  "<t4>"
  Bus Selector/5 -> t5/1  "<t5>"
  Bus Selector/6 -> t6/1  "<t6>"
  t/1 -> Bus Selector/1
